simulink model "GenerateIPMSMCurrentProfile"  (R2026a)
settings: Solver=FixedStepAuto  StopTime=0.01  FixedStep=Ts
PreLoadFcn:
  | load('Model_Init.mat');
values from neighbouring files (symbols this model uses):
  BW = 750    [Model_Init.mat]
  idAxis = [-900 -882 -864 -846 -828 -810 -792 -774 -756 -738 -720 -702 ... (51 elements, 1x51)]    [Model_Init.mat]
  iqAxis = [0 17.3076923077 34.6153846154 51.9230769231 69.2307692308 86.5384615385 103.846153846 121.153846154 138.461538462 155.769230769 173.076923077 190.384615385 ... (53 elements, 1x53)]    [Model_Init.mat]
  Ki_d = 74.9060598039    [Model_Init.mat]
  Ki_q = 74.9060598039    [Model_Init.mat]
  lambdad = [-0.0631189178304 -0.0604505535566 -0.0577660230755 -0.0550656704567 -0.0523339959385 -0.0495630530333 -0.0467724011475 -0.043961149999 -0.041088360542 -0.0381850897745 -0.0352575152962 -0.0322924487897 ... (2703 elements, 51x53)]    [Model_Init.mat]
  lambdaq = [1.81058605777e-05 1.90263877371e-05 1.96027346878e-05 2.01239748193e-05 2.12091984783e-05 2.18705193678e-05 2.23125714149e-05 2.2585012385e-05 2.28163786723e-05 2.26620263018e-05 2.21885293033e-05 2.13315493573e-05 ... (2703 elements, 51x53)]    [Model_Init.mat]
  Ldd = [0.000148242459653 0.000148691520968 0.000149580086108 0.000150889642696 0.000152850483985 0.000154488744193 0.000155608417618 0.00015789001682 0.000160446117349 0.000161967923494 0.0001636844718 0.000166282231015 ... (2703 elements, 51x53)]    [Model_Init.mat]
  Lqq = [0.000400557309226 0.000405173323325 0.000409987177942 0.000414914340273 0.000419888602874 0.000424960583757 0.000430114747461 0.000435342158236 0.000440633705793 0.000446010815939 0.000451479502648 0.000457041392507 ... (2703 elements, 51x53)]    [Model_Init.mat]
  optimalTables =     [Model_Init.mat]
  PolePairs = 4    [Model_Init.mat]
  Ts = 1e-06    [Model_Init.mat]
  Tst = 0.0001    [Model_Init.mat]
undefined symbols (not defined in the file or in its folder): DiscIntNeverNeededParam
libraries: nesl_utility x13, fl_lib x7, ee_lib x5, eePwmGeneratorTwoLevel x1
settings Model: Creator=dakaihu  LastModifiedBy=dakaihu
settings SimscapeCC: SimscapeNominalValues="[{\"value\":\"1\",\"unit\":\"A\"},{\"value\":\"1\",\"unit\":\"bar\"},{\"value\":\"1\",\"unit\":\"cm^2\"},{\"value\":\"1\",\"unit\":\"cm^3/s\"},{\"value\":\"1\",\"unit\":\"kJ/kg\"},{\"value\":\"1\",\"unit\":\"kW\"},{\"value\":\"1\",\"unit\":\"l\"},{\"value\":\"1\",\"unit\":\"N\"},{\"value\":\"1\",\"unit\":\"N*m\"},{\"value\":\"1\",\"unit\":\"V\"}]"  SimscapeLogType=none  SimscapeLogDataHistory=5000.0

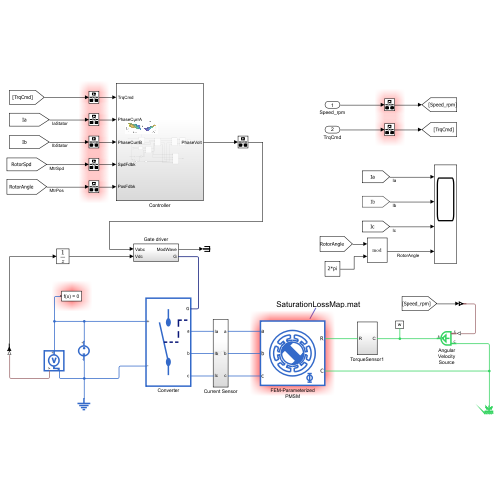
[thumbnail: Simulink's stored preview of the top-level diagram]
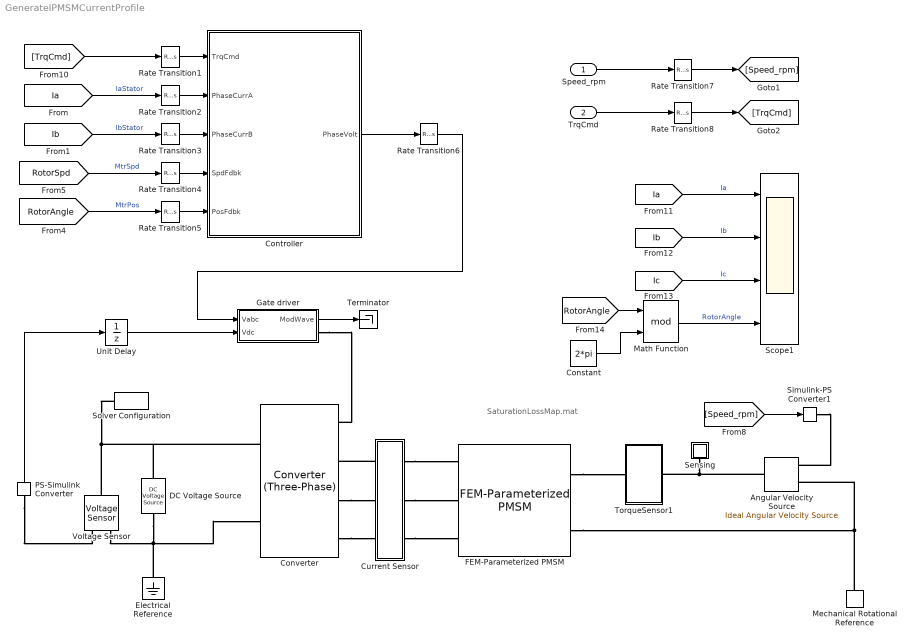
== system GenerateIPMSMCurrentProfile ==
  note: SaturationLossMap.mat
  Speed_rpm : Inport
  TrqCmd : Inport  Port=2
  Angular Velocity Source : fl_lib/Mechanical/Mechanical Sources/Ideal Angular Velocity Source
  Constant : Constant  Value=2*pi
  Controller : Subsystem
  Converter : ee_lib/Semiconductors & Converters/Converters/Converter (Three-Phase)  port_option=ee.enum.threePhasePort.expanded  fidelity_option=ee.enum.converters.fidelity.detailed  device_type=3  showThermalPort=false  K=0  Vth=0.5 V  Vgt=1 V  Vgt_off=-1 V  Ih=1 A  Vf=0.8 V  Ron=0.001 Ohm  Rds=0.001 Ohm  Goff=1e-5 1/Ohm  Eon_scalar=22.86e-3 J  Eoff_scalar=17.14e-3 J  Eoff_natural_commutation=10e-3 J  Voff=300 V  Iout_scalar=600 A  onCurrentMeasDelay=0 s  useCurrentFromPreviousCycle=false  useVoltageFromPreviousCycle=false  diode_param=2  diode_Vf=0.8 V  diode_Ron=0.001 Ohm  diode_Goff=1e-5 1/Ohm  diode_C=50 nF  diode_iRM=-235 A  diode_iF=300 A  diode_idot=-50 A/us  diode_trr_param=1  diode_trr_factor=3  diode_trr=15 us  diode_Qrr=1.5e+3 s*uA  diode_rec_loss_model=ee.enum.diode.reverseRecoveryModel.fixed  diode_ErecVal=0 J  diode_scaleWithIandV=false  diode_ErecMat=zeros(2, 3) J  diode_TjrecVec=[298.15, 398.15] K  diode_IfrecVec=[.1, 1, 10] A  diode_IrecVal=10 A  diode_VrecVal=10 V  diode_tFilter=1 / 1000 / 100 s  thermal_network_parameterization=ee.enum.thermalNetworkTopology.external  Rth=[.08, .5] K/W  Rth_Cauer=[.08, .1, .5] K/W  Rth_Foster=[.08, .14, .22, .16] K/W  thermal_mass_parameterization=ee.enum.thermalNetwork.timeconstant  thermal_mass=[.01, .5] J/K  thermal_mass_Cauer=[.01, .1, .5] J/K  thermal_mass_Foster=[.001, .005, .05, .5] J/K  thermal_time_constant=[.001, .2] s  thermal_time_constant_Cauer=[.001, .1, .2] s  thermal_time_constant_Foster=[7e-05, .0007, .01, .08] s  thermal_mass_initial_temperatures=[25, 25] degC  thermal_mass_initial_temperatures_Cauer=[25, 25, 25] degC  junction_thermal_mass=0.01 J/K  Tvec_initial_Foster=[25, 25, 25, 25] degC  snubber_type=0  Cs=1e-7 F  Rs=0.1 Ohm  Vce_loss=[0, 150, 300] V
  Current Sensor : Subsystem
  DC Voltage Source : ee_lib/Additional Components/SPICE Sources/DC Voltage Source  DC=720 V
  Electrical Reference : fl_lib/Electrical/Electrical Elements/Electrical Reference
  FEM-Parameterized PMSM : ee_lib/Electromechanical/Permanent Magnet/FEM-Parameterized PMSM  parameterization=1  winding_type=ee.enum.statorconnection.wye  iVec=[-2, 0, 2] A  xVec=[0, 20, 40, 60] deg  dfluxdiMatrix=0.0002 * ones(3, 4) Wb/A  dfluxdxMatrix=[0, -.16, .16, 0; 0, -.16, .16, 0; 0, -.16, .16, 0] Wb/rad  calculate_torque_matrix=1  TorqueMatrix=zeros(3, 3, 3, 4) N*m  idVec1=[-200, 0, 200] A  iqVec1=[-200, 0, 200] A  LdMatrix=0.0002 * ones(3, 3) H  LqMatrix=0.0002 * ones(3, 3) H  PmMatrix=0.1 * ones(3, 3) Wb  interp_method=simscape.enum.interpolation.linear  N=6  Rs=Rs Ohm  Ms=0.00002 H  L0=0.00016 H  loss_param=ee.enum.fem_motor.ironLossesExtended.empirical  losses_oc=[0, 0, 0] W  losses_sc=[0, 0, 0] W  f_losses=60 Hz  Isc_losses=95 A  Inertia=0 kg*m^2  lam=0 N*m/(rad/s)  i_d_specify=off  i_d_priority=None  i_d=0 A  i_d_nominal_specify=off  i_d_nominal_value=1  i_d_nominal_unit=A  i_q_specify=off  i_q_priority=None  i_q=0 A  i_q_nominal_specify=off  i_q_nominal_value=1  i_q_nominal_unit=A  torque_specify=off  torque_priority=None  torque=0 N*m  torque_nominal_specify=off  torque_nominal_value=1  torque_nominal_unit=N*m  angular_velocity_specify=on  angular_velocity_priority=Low  angular_velocity=1000 rpm  angular_velocity_nominal_specify=off  angular_velocity_nominal_value=1  angular_velocity_nominal_unit=rpm  angular_position_specify=off  angular_position_priority=High  angular_position=0 deg  angular_position_nominal_specify=off  angular_position_nominal_value=1  angular_position_nominal_unit=deg  alpha=3.93e-3 1/K  alpha_flux=-0.001 1/K  Tmeas=298.15 K  stator_thermal_mass=100 J/K  stator_initial_temperatures=[298.15, 298.15, 298.15] K  rotor_thermal_mass=200 J/K  rotor_initial_temperature=298.15 K  Rm_percent_rotor=90  Rd_percent_rotor=30  idVec=[-200, 0, 200] A  iqVec=[-200, 0, 200] A  dfluxAdiaMatrix3D=zeros(3, 3, 4) Wb/A  dfluxAdibMatrix3D=zeros(3, 3, 4) Wb/A  dfluxAdicMatrix3D=zeros(3, 3, 4) Wb/A  dfluxAdxMatrix3D=zeros(3, 3, 4) Wb/rad  TorqueMatrix3D=zeros(3, 3, 4) N*m  iaVec=[-200, 0, 200] A  ibVec=[-200, 0, 200] A  icVec=[-200, 0, 200] A  dfluxAdiaMatrix=zeros(3, 3, 3, 4) Wb/A  dfluxAdibMatrix=zeros(3, 3, 3, 4) Wb/A  dfluxAdicMatrix=zeros(3, 3, 3, 4) Wb/A  dfluxAdxMatrix=zeros(3, 3, 3, 4) Wb/rad  param_dq0=ee.enum.fem_motor.fluxTabulationOption.DQpolar  winding_type_dq0=1  expose_neutral_port=ee.enum.fem_motor.exposeNeutralPort.no  nPolePairs=PolePairs  parks_type=ee.enum.fem_motor.parksType.QleadsD_AphaseToQaxis  idVec2=idVec A  iqVec2=iqVec A  magVec2=MagVec A  betaVec2=gammaVec deg  xVec2=angleVec deg  fluxD_dq0=fluxD Wb  fluxQ_dq0=fluxQ Wb  fluxA_dq0=fluxAmat Wb  Torque_dq0=torque N*m  fluxD_IBX=Fd Wb  fluxQ_IBX=Fq Wb  fluxA_IBX=fluxAmat Wb  Torque_IBX=torqueMat N*m  rotorLossCoeff_k_h_DQ=zeros(3, 3) W/Hz  rotorLossCoeff_k_J_DQ=zeros(3, 3) W/Hz^2  rotorLossCoeff_k_ex_DQ=zeros(3, 3) W/Hz^1.50000  rotorLossCoeff_k_h_IB=zeros(3, 5) W/Hz  rotorLossCoeff_k_J_IB=zeros(3, 5) W/Hz^2  rotorLossCoeff_k_ex_IB=zeros(3, 5) W/Hz^1.50000  statorLossCoeff_k_h_DQ=zeros(3, 3) W/Hz  statorLossCoeff_k_J_DQ=zeros(3, 3) W/Hz^2  statorLossCoeff_k_ex_DQ=zeros(3, 3) W/Hz^1.50000  statorLossCoeff_k_h_IB=zeros(3, 5) W/Hz  statorLossCoeff_k_J_IB=zeros(3, 5) W/Hz^2  statorLossCoeff_k_ex_IB=zeros(3, 5) W/Hz^1.50000  wVec=[1000, 2000] rpm  rotorLossTable_DQ=zeros(3, 3, 2) W  statorLossTable_DQ=zeros(3, 3, 2) W  rotorLossTable_IB=zeros(3, 5, 2) W  statorLossTable_IB=zeros(3, 5, 2) W  electrical_torque_before_iron_losses_specify=off  electrical_torque_before_iron_losses_priority=None  electrical_torque_before_iron_losses=0 N*m  electrical_torque_before_iron_losses_nominal_specify=off  electrical_torque_before_iron_losses_nominal_value=1  electrical_torque_before_iron_losses_nominal_unit=N*m  Qrotor_specify=off  Qrotor_priority=None  Qrotor=0 J/s  Qrotor_nominal_specify=off  Qrotor_nominal_value=1  Qrotor_nominal_unit=J/s  Qstator_specify=off  Qstator_priority=None  Qstator=0 J/s  Qstator_nominal_specify=off  Qstator_nominal_value=1  Qstator_nominal_unit=J/s
  Gate driver : Subsystem
  Math Function : Math  Operator=mod
  Mechanical Rotational Reference : fl_lib/Mechanical/Rotational Elements/Mechanical Rotational Reference
  PS-Simulink Converter : nesl_utility/PS-Simulink Converter  PhysicalDomain=network_engine_domain  SubClassName=ps_output  LeftPortType=input  RightPortType=output  PseudoPeriodic=off  Frequencies=[]  VectorFormat=inherit  Unit=V  AffineConversion=off
  Rate Transition{1..5,7..8} (7 alike) : RateTransition  OutPortSampleTime=Tst
  Rate Transition6 : RateTransition
  Scope1 : Scope  NumInputPorts=4
      settings: ActiveDisplayYMinimum=-1.2392913585991725E-13  ActiveDisplayYMaximum=1.093469821040979E-12  DataLoggingVariableName=IPMSM_Currents  DataLoggingSaveFormat=Structure
  Sensing : Subsystem
      mask Display: disp('w');
  Simulink-PS Converter1 : nesl_utility/Simulink-PS Converter  PhysicalDomain=network_engine_domain  SubClassName=ps_input  LeftPortType=input  RightPortType=output  PseudoPeriodic=off  Frequencies=[]  NoiseDistribution=none  NoiseParameters=[]  Unit=rpm  AffineConversion=off  FilteringAndDerivatives=provide  SimscapeFilterOrder=1  InputFilterTimeConstant=0.001  UdotUserProvided=0
  Solver Configuration : nesl_utility/Solver Configuration  PhysicalDomain=network_engine_domain  SubClassName=solver  LeftPortType=input  RightPortType=generic  Tones=[]  Harmonics=[]  SimulateNoise=off  Profile=off  UseLocalSampling=off  EnableSwitchedLinearOptims=on  FrequencyDomain=off  UseCCode=off  RelTol=0.001  AbsTol=1e-06  MinStep=1e-09  ToWorkspace=off  RevertToSquareIcSolve=off  NumHomotopyIterations=100  PhasorMode=off  PhasorModeNumHarmonics=1  ConsistencySolver=NEWTON_FTOL  CanonicalOrdering=UNORDERED  OptimizeIntermediates=UNOPTIMIZED  IndexReductionMethod=DerivativeReplacement  DoDC=off  ResidualTolerance=1e-9  ConsistencyTolSource=GLOBAL  ConsistencyAbsTol=0.001  ConsistencyRelTol=0.001  ConsistencyTolFactor=0.001  UseLocalSolver=on  LocalSolverChoice=NE_BACKWARD_EULER_ADVANCER  ResolveIndetEquations=on  FunctionEvalNumThread=1  LocalSolverSampleTime=Ts  DoFixedCost=off  MaxNonlinIter=4  MaxModeIter=2  ComputeImpulses=off  ImpulseIterations=2  LinearAlgebra=auto  LinearAlgebraNumThread=0  EquationFormulation=NE_TIME_EF  DelaysMemoryBudget=1024  AutomaticFiltering=on  FilteringTimeConstant=0.001  PartitionStorageMethod=AS_NEEDED  PartitionMemoryBudget=1024  PartitionMethod=FAST  MultibodyUseLocalSolver=off  MultibodyLocalSolverChoice=ODE1  MultibodyLocalSolverSampleTime=0.001
  Terminator : Terminator
  TorqueSensor1 : Subsystem
  Unit Delay : UnitDelay  SampleTime=-1
  Voltage Sensor : fl_lib/Electrical/Electrical Sensors/Voltage Sensor
  wires:
  Controller/1(PhaseVolt) -> Rate Transition6/1
  [TrqCmd] -> Rate Transition1/1
  [Ia] -> Rate Transition2/1  "IaStator"
  [RotorSpd] -> Rate Transition4/1  "MtrSpd"
  [RotorAngle] -> Rate Transition5/1  "MtrPos"
  Rate Transition1/1 -> Controller/1(TrqCmd)
  Rate Transition2/1 -> Controller/2(PhaseCurrA)
  [Ib] -> Rate Transition3/1  "IbStator"
  Rate Transition3/1 -> Controller/3(PhaseCurrB)
  Rate Transition4/1 -> Controller/4(SpdFdbk)
  Rate Transition5/1 -> Controller/5(PosFdbk)
  Rate Transition6/1 -> Gate driver/1(Vabc)
  Unit Delay/1 -> Gate driver/2(Vdc)
  Gate driver/1(ModWave) -> Terminator/1
  [Speed_rpm] -> Simulink-PS Converter1/1
  PS-Simulink Converter/1 -> Unit Delay/1
  Rate Transition7/1 -> [Speed_rpm]
  Rate Transition8/1 -> [TrqCmd]
  [RotorAngle] -> Math Function/1
  Constant/1 -> Math Function/2
  [Ia] -> Scope1/1  "Ia"
  [Ib] -> Scope1/2  "Ib"
  [Ic] -> Scope1/3  "Ic"
  Math Function/1 -> Scope1/4  "RotorAngle"
  Speed_rpm/1 -> Rate Transition7/1
  TrqCmd/1 -> Rate Transition8/1
  connections:
  Sensing/LConn1 -- Angular Velocity Source/LConn1 -- TorqueSensor1/RConn1
  Mechanical Rotational Reference/LConn1 -- Angular Velocity Source/RConn2 -- FEM-Parameterized PMSM/RConn2
  Solver Configuration/RConn1 -- Converter/RConn1 -- DC Voltage Source/LConn1 -- Voltage Sensor/LConn1
  Electrical Reference/LConn1 -- Converter/RConn2 -- DC Voltage Source/RConn1 -- Voltage Sensor/RConn2
  Gate driver/RConn1 -- Converter/LConn1
  Current Sensor/LConn1 -- Converter/LConn2
  Current Sensor/RConn1 -- FEM-Parameterized PMSM/LConn1
  Converter/LConn3 -- Current Sensor/LConn2
  Current Sensor/RConn2 -- FEM-Parameterized PMSM/LConn2
  Converter/LConn4 -- Current Sensor/LConn3
  Current Sensor/RConn3 -- FEM-Parameterized PMSM/LConn3
  Simulink-PS Converter1/RConn1 -- Angular Velocity Source/RConn1
  PS-Simulink Converter/LConn1 -- Voltage Sensor/RConn1
  FEM-Parameterized PMSM/RConn1 -- TorqueSensor1/LConn1

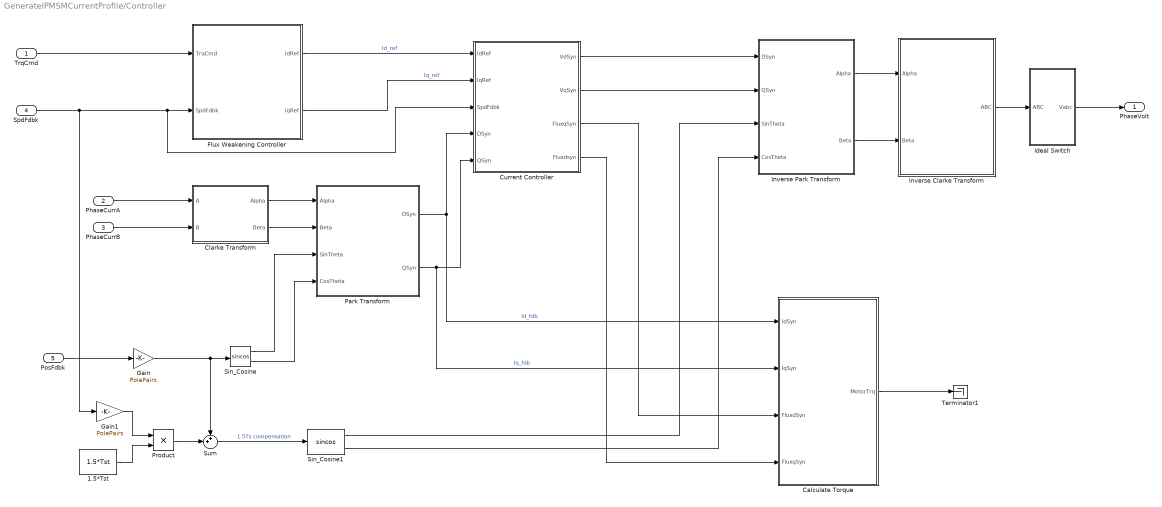
== system GenerateIPMSMCurrentProfile/Controller ==
  TrqCmd : Inport  OutDataTypeStr=double  PortDimensions=1  SampleTime=Tst
  PhaseCurrA : Inport  Port=2  OutDataTypeStr=double  PortDimensions=1  SampleTime=Tst
  PhaseCurrB : Inport  Port=3  OutDataTypeStr=double  PortDimensions=1  SampleTime=Tst
  SpdFdbk : Inport  Port=4  OutDataTypeStr=double  PortDimensions=1  SampleTime=Tst
  PosFdbk : Inport  Port=5  OutDataTypeStr=double  PortDimensions=1  SampleTime=Tst
  1.5*Tst : Constant  Value=1.5*Tst  SampleTime=-1
  Calculate Torque : Subsystem
  Clarke Transform : Subsystem
  Current Controller : Subsystem
  Flux Weakening Controller : Subsystem
  Gain : Gain  Gain=PolePairs
  Gain1 : Gain  Gain=PolePairs
  Ideal Switch : Subsystem  VariantControl=SpaceVectorModulation_JB
  Inverse Clarke Transform : Subsystem
  Inverse Park Transform : Subsystem
  Park Transform : Subsystem
  Product : Product
  Sin_Cosine : Trigonometry  Operator=sincos
  Sin_Cosine1 : Trigonometry  Operator=sincos
  Sum : Sum  Inputs=++|
  Terminator1 : Terminator
  PhaseVolt : Outport  OutDataTypeStr=double  Unit=V  PortDimensions=3  SampleTime=Tst  VectorParamsAs1DForOutWhenUnconnected=off
  wires:
  Flux Weakening Controller/1(IdRef) -> Current Controller/1(IdRef)  "Id_ref"
  SpdFdbk/1 -> Gain1/1, Current Controller/3(SpdFdbk), Flux Weakening Controller/2(SpdFdbk)
  Gain1/1 -> Product/1
  Sum/1 -> Sin_Cosine1/1  "1.5Ts compensation"
  Clarke Transform/1(Alpha) -> Park Transform/1(Alpha)
  Clarke Transform/2(Beta) -> Park Transform/2(Beta)
  Current Controller/1(VdSyn) -> Inverse Park Transform/1(DSyn)
  Inverse Park Transform/1(Alpha) -> Inverse Clarke Transform/1(Alpha)
  Sin_Cosine/1 -> Park Transform/3(SinTheta)
  Park Transform/2(QSyn) -> Current Controller/5(QSyn), Calculate Torque/2(IqSyn)  "Iq_fdb"
  Product/1 -> Sum/2
  Sin_Cosine/2 -> Park Transform/4(CosTheta)
  1.5*Tst/1 -> Product/2
  Calculate Torque/1(MotorTrq) -> Terminator1/1
  Current Controller/2(VqSyn) -> Inverse Park Transform/2(QSyn)
  Current Controller/3(FluxqSyn) -> Calculate Torque/3(FluxdSyn)
  Inverse Clarke Transform/1(ABC) -> Ideal Switch/1(ABC)
  PosFdbk/1 -> Gain/1
  Inverse Park Transform/2(Beta) -> Inverse Clarke Transform/2(Beta)
  Gain/1 -> Sum/1, Sin_Cosine/1
  PhaseCurrB/1 -> Clarke Transform/2(B)
  Park Transform/1(DSyn) -> Current Controller/4(DSyn), Calculate Torque/1(IdSyn)  "Id_fdb"
  TrqCmd/1 -> Flux Weakening Controller/1(TrqCmd)
  Current Controller/4(Fluxdsyn) -> Calculate Torque/4(FluxqSyn)
  Flux Weakening Controller/2(IqRef) -> Current Controller/2(IqRef)  "Iq_ref"
  Sin_Cosine1/2 -> Inverse Park Transform/4(CosTheta)
  Sin_Cosine1/1 -> Inverse Park Transform/3(SinTheta)
  PhaseCurrA/1 -> Clarke Transform/1(A)
  Ideal Switch/1(Vabc) -> PhaseVolt/1

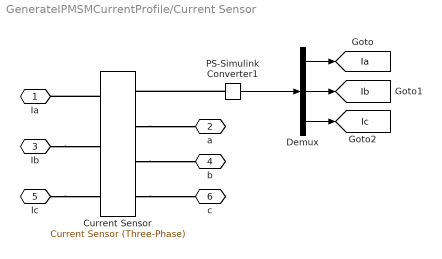
== system GenerateIPMSMCurrentProfile/Current Sensor ==
  Current Sensor : ee_lib/Sensors & Transducers/Current Sensor (Three-Phase)  port_option=ee.enum.threePhasePort.expanded
  Demux : Demux  Outputs=3
  PS-Simulink Converter1 : nesl_utility/PS-Simulink Converter  PhysicalDomain=network_engine_domain  SubClassName=ps_output  LeftPortType=input  RightPortType=output  PseudoPeriodic=off  Frequencies=[]  VectorFormat=inherit  Unit=A  AffineConversion=off
  Ia : PMIOPort  Side=Left
  a : PMIOPort  Port=2  Side=Right
  Ib : PMIOPort  Port=3  Side=Left
  b : PMIOPort  Port=4  Side=Right
  Ic : PMIOPort  Port=5  Side=Left
  c : PMIOPort  Port=6  Side=Right
  tag scope: Ia=global, Ib=global, Ic=global
  wires:
  Demux/1 -> [Ia]
  Demux/2 -> [Ib]
  Demux/3 -> [Ic]
  PS-Simulink Converter1/1 -> Demux/1
  connections:
  Current Sensor/RConn3 -- b/RConn1
  Ib/RConn1 -- Current Sensor/LConn2
  Current Sensor/RConn2 -- a/RConn1
  Current Sensor/LConn1 -- Ia/RConn1
  Current Sensor/RConn4 -- c/RConn1
  Ic/RConn1 -- Current Sensor/LConn3
  PS-Simulink Converter1/LConn1 -- Current Sensor/RConn1

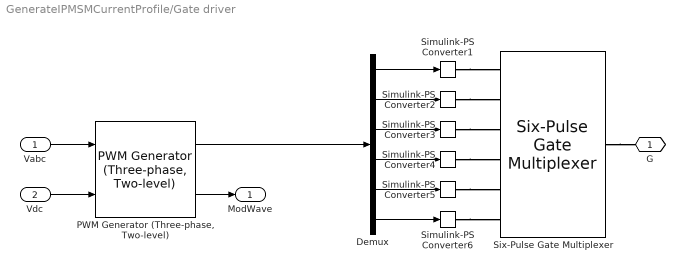
== system GenerateIPMSMCurrentProfile/Gate driver ==
  Vabc : Inport
  Vdc : Inport  Port=2
  Demux : Demux  Outputs=6
  "PWM Generator (Three-phase, Two-level)" : eePwmGeneratorTwoLevel/PWM Generator (Three-phase, Two-level)  PWMMode=Continuous PWM (CPWM)  CPWMMode=SVM: space vector modulation  DPWMMode=60 DPWM: 60 degree discontinuous PWM  fsw=1e4  Ts=Ts
  Simulink-PS Converter{1..6} (6 alike) : nesl_utility/Simulink-PS Converter  PhysicalDomain=network_engine_domain  SubClassName=ps_input  LeftPortType=input  RightPortType=output  PseudoPeriodic=off  Frequencies=[]  NoiseDistribution=none  NoiseParameters=[]  Unit=1  AffineConversion=off  FilteringAndDerivatives=zero  SimscapeFilterOrder=1  InputFilterTimeConstant=0.001  UdotUserProvided=1
  Six-Pulse Gate Multiplexer : ee_lib/Semiconductors & Converters/Converters/Six-Pulse Gate Multiplexer  port_option=ee.enum.controlport.ps
  G : PMIOPort  Side=Right
  ModWave : Outport
  wires:
  Demux/2 -> Simulink-PS Converter2/1
  Demux/3 -> Simulink-PS Converter3/1
  Demux/4 -> Simulink-PS Converter4/1
  Demux/6 -> Simulink-PS Converter6/1
  Demux/5 -> Simulink-PS Converter5/1
  "PWM Generator (Three-phase, Two-level)"/1 -> Demux/1
  Demux/1 -> Simulink-PS Converter1/1
  "PWM Generator (Three-phase, Two-level)"/2 -> ModWave/1
  Vdc/1 -> "PWM Generator (Three-phase, Two-level)"/2
  Vabc/1 -> "PWM Generator (Three-phase, Two-level)"/1
  connections:
  Simulink-PS Converter4/RConn1 -- Six-Pulse Gate Multiplexer/LConn4
  Simulink-PS Converter3/RConn1 -- Six-Pulse Gate Multiplexer/LConn3
  Simulink-PS Converter2/RConn1 -- Six-Pulse Gate Multiplexer/LConn2
  Simulink-PS Converter6/RConn1 -- Six-Pulse Gate Multiplexer/LConn6
  Simulink-PS Converter5/RConn1 -- Six-Pulse Gate Multiplexer/LConn5
  Simulink-PS Converter1/RConn1 -- Six-Pulse Gate Multiplexer/LConn1
  Six-Pulse Gate Multiplexer/RConn1 -- G/RConn1

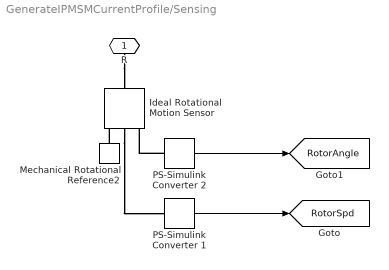
== system GenerateIPMSMCurrentProfile/Sensing ==
  Ideal Rotational Motion Sensor : fl_lib/Mechanical/Mechanical Sensors/Ideal Rotational Motion Sensor  reference=foundation.enum.MeasurementReference.difference  acceleration_port=false  velocity_port=true  position_port=true  wrap_angle=simscape.enum.onoff.off  offset=0 rad
  Mechanical Rotational Reference2 : fl_lib/Mechanical/Rotational Elements/Mechanical Rotational Reference
  PS-Simulink Converter 1 : nesl_utility/PS-Simulink Converter  PhysicalDomain=network_engine_domain  SubClassName=ps_output  LeftPortType=input  RightPortType=output  PseudoPeriodic=off  Frequencies=[]  VectorFormat=1-D array  Unit=rad/s  AffineConversion=off
  PS-Simulink Converter 2 : nesl_utility/PS-Simulink Converter  PhysicalDomain=network_engine_domain  SubClassName=ps_output  LeftPortType=input  RightPortType=output  PseudoPeriodic=off  Frequencies=[]  VectorFormat=1-D array  Unit=rad  AffineConversion=off
  R : PMIOPort  Side=Left
  tag scope: RotorAngle=global, RotorSpd=global
  wires:
  PS-Simulink Converter 1/1 -> [RotorSpd]
  PS-Simulink Converter 2/1 -> [RotorAngle]
  connections:
  Ideal Rotational Motion Sensor/RConn2 -- PS-Simulink Converter 1/LConn1
  Mechanical Rotational Reference2/LConn1 -- Ideal Rotational Motion Sensor/RConn1
  R/RConn1 -- Ideal Rotational Motion Sensor/LConn1
  PS-Simulink Converter 2/LConn1 -- Ideal Rotational Motion Sensor/RConn3

== system GenerateIPMSMCurrentProfile/TorqueSensor1 ==
  Goto11 : Goto  Commented=on  GotoTag=MotorTrq  TagVisibility=global
  Ideal Torque Sensor1 : fl_lib/Mechanical/Mechanical Sensors/Ideal Torque Sensor
  PS-Simulink Converter1 : nesl_utility/PS-Simulink Converter  PhysicalDomain=network_engine_domain  SubClassName=ps_output  LeftPortType=input  RightPortType=output  PseudoPeriodic=off  Frequencies=[]  VectorFormat=inherit  Unit=N*m  AffineConversion=off
  R : PMIOPort  Side=Left
  C : PMIOPort  Port=2  Side=Right
  wires:
  PS-Simulink Converter1/1 -> Goto11/1
  connections:
  Ideal Torque Sensor1/RConn2 -- PS-Simulink Converter1/LConn1
  R/RConn1 -- Ideal Torque Sensor1/LConn1
  C/RConn1 -- Ideal Torque Sensor1/RConn1

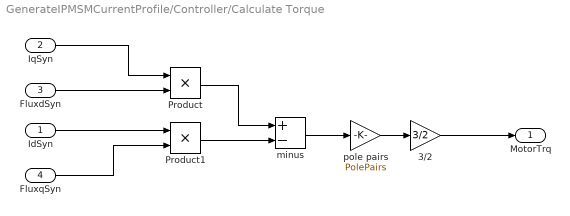
== system GenerateIPMSMCurrentProfile/Controller/Calculate Torque ==
  IdSyn : Inport
  IqSyn : Inport  Port=2
  FluxdSyn : Inport  Port=3
  FluxqSyn : Inport  Port=4
  3/2 : Gain  Gain=3/2
  Product : Product
  Product1 : Product
  minus : Sum  Inputs=+-
  pole pairs : Gain  Gain=PolePairs
  MotorTrq : Outport  VectorParamsAs1DForOutWhenUnconnected=off
  wires:
  FluxqSyn/1 -> Product1/2
  FluxdSyn/1 -> Product/2
  pole pairs/1 -> 3/2/1
  IdSyn/1 -> Product1/1
  IqSyn/1 -> Product/1
  Product/1 -> minus/1
  minus/1 -> pole pairs/1
  Product1/1 -> minus/2
  3/2/1 -> MotorTrq/1

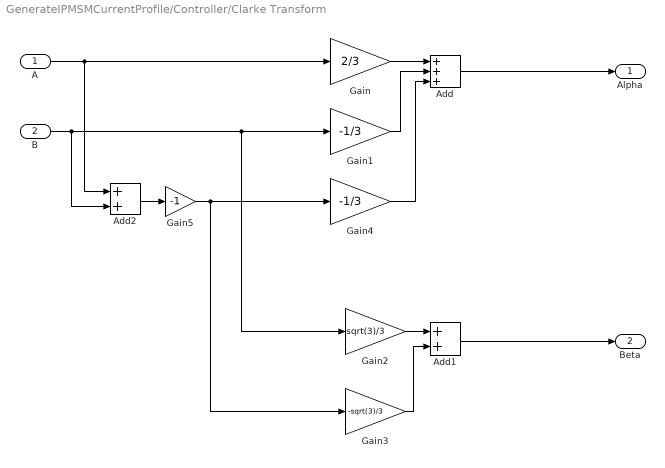
== system GenerateIPMSMCurrentProfile/Controller/Clarke Transform ==
  A : Inport
  B : Inport  Port=2
  Add : Sum  Inputs=+++
  Add1 : Sum
  Add2 : Sum
  Gain : Gain  Gain=2/3
  Gain1 : Gain  Gain=-1/3
  Gain2 : Gain  Gain=sqrt(3)/3
  Gain3 : Gain  Gain=-sqrt(3)/3
  Gain4 : Gain  Gain=-1/3
  Gain5 : Gain  Gain=-1
  Alpha : Outport  VectorParamsAs1DForOutWhenUnconnected=off
  Beta : Outport  Port=2  VectorParamsAs1DForOutWhenUnconnected=off
  wires:
  Gain5/1 -> Gain3/1, Gain4/1
  A/1 -> Gain/1, Add2/1
  Gain/1 -> Add/1
  B/1 -> Gain2/1, Gain1/1, Add2/2
  Gain1/1 -> Add/2
  Add/1 -> Alpha/1
  Add1/1 -> Beta/1
  Gain2/1 -> Add1/1
  Add2/1 -> Gain5/1
  Gain3/1 -> Add1/2
  Gain4/1 -> Add/3

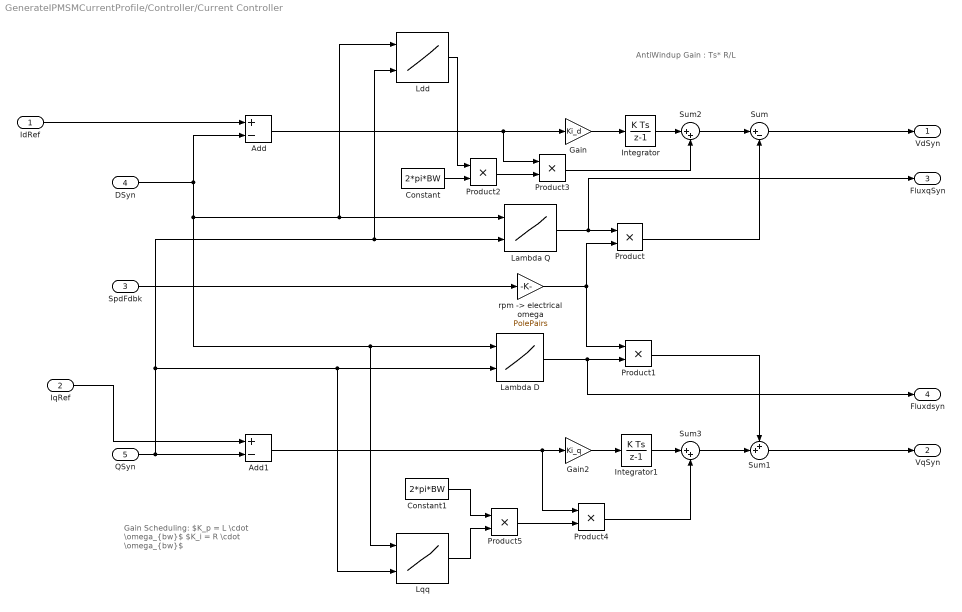
== system GenerateIPMSMCurrentProfile/Controller/Current Controller ==
  note: AntiWindup Gain : Ts* R/L
  note: Gain Scheduling:
      | $K_p = L \cdot \omega_{bw}$
      | $K_i = R \cdot \omega_{bw}$
  IdRef : Inport
  IqRef : Inport  Port=2
  SpdFdbk : Inport  Port=3
  DSyn : Inport  Port=4
  QSyn : Inport  Port=5
  Add : Sum  Inputs=+-
  Add1 : Sum  Inputs=+-
  Constant : Constant  Value=2*pi*BW  SampleTime=-1
  Constant1 : Constant  Value=2*pi*BW  SampleTime=-1
  Gain : Gain  Gain=Ki_d
  Gain2 : Gain  Gain=Ki_q
  Integrator : DiscreteIntegrator  SampleTime=-1  ICPrevOutput=DiscIntNeverNeededParam  ICPrevScaledInput=DiscIntNeverNeededParam
  Integrator1 : DiscreteIntegrator  SampleTime=-1  ICPrevOutput=DiscIntNeverNeededParam  ICPrevScaledInput=DiscIntNeverNeededParam
  Lambda D : Lookup_n-D  BreakpointsForDimension1=idAxis  BreakpointsForDimension2=iqAxis  BreakpointsForDimension3=[5, 7]  Table=lambdad  InternalRulePriority=Speed  RndMeth=Simplest
      settings: InputPortMap=u0,u1
  Lambda Q : Lookup_n-D  BreakpointsForDimension1=idAxis  BreakpointsForDimension2=iqAxis  BreakpointsForDimension3=[5, 7]  Table=lambdaq  InternalRulePriority=Speed  RndMeth=Simplest
      settings: InputPortMap=u0,u1
  Ldd : Lookup_n-D  BreakpointsForDimension1=idAxis  BreakpointsForDimension2=iqAxis  BreakpointsForDimension3=[5, 7]  Table=Ldd  InternalRulePriority=Speed  RndMeth=Simplest
      settings: InputPortMap=u0,u1
  Lqq : Lookup_n-D  BreakpointsForDimension1=idAxis  BreakpointsForDimension2=iqAxis  BreakpointsForDimension3=[5, 7]  Table=Lqq  InternalRulePriority=Speed  RndMeth=Simplest
      settings: InputPortMap=u0,u1
  Product{,1..5} (6 alike) : Product
  Sum : Sum  Inputs=|+-
  Sum1 : Sum  Inputs=++|
  Sum2 : Sum  Inputs=|++
  Sum3 : Sum  Inputs=|++
  "rpm -> electrical omega" : Gain  Gain=PolePairs
  VdSyn : Outport  VectorParamsAs1DForOutWhenUnconnected=off
  VqSyn : Outport  Port=2  VectorParamsAs1DForOutWhenUnconnected=off
  FluxqSyn : Outport  Port=3  VectorParamsAs1DForOutWhenUnconnected=off
  Fluxdsyn : Outport  Port=4  VectorParamsAs1DForOutWhenUnconnected=off
  wires:
  Add1/1 -> Product4/1, Gain2/1
  Sum3/1 -> Sum1/2
  Product4/1 -> Sum3/2
  Gain2/1 -> Integrator1/1
  Integrator1/1 -> Sum3/1
  Sum2/1 -> Sum/1
  Add/1 -> Product3/1, Gain/1
  Product3/1 -> Sum2/2
  Integrator/1 -> Sum2/1
  Gain/1 -> Integrator/1
  Sum1/1 -> VqSyn/1
  Sum/1 -> VdSyn/1
  Product1/1 -> Sum1/1
  Lambda D/1 -> Product1/2, Fluxdsyn/1
  DSyn/1 -> Add/2, Ldd/1, Lambda Q/1, Lambda D/1, Lqq/1
  QSyn/1 -> Add1/2, Lqq/2, Lambda D/2, Ldd/2, Lambda Q/2
  "rpm -> electrical omega"/1 -> Product/2, Product1/1
  Lambda Q/1 -> Product/1, FluxqSyn/1
  IqRef/1 -> Add1/1
  SpdFdbk/1 -> "rpm -> electrical omega"/1
  IdRef/1 -> Add/1
  Ldd/1 -> Product2/1
  Constant/1 -> Product2/2
  Product2/1 -> Product3/2
  Product5/1 -> Product4/2
  Constant1/1 -> Product5/1
  Lqq/1 -> Product5/2
  Product/1 -> Sum/2

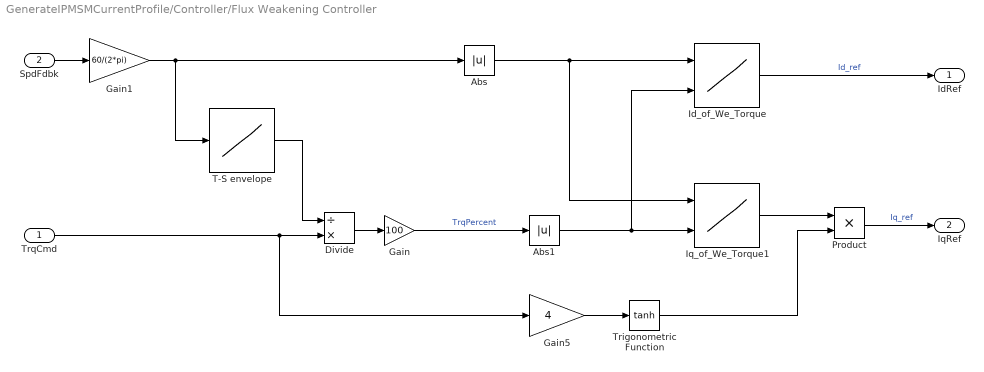
== system GenerateIPMSMCurrentProfile/Controller/Flux Weakening Controller ==
  TrqCmd : Inport
  SpdFdbk : Inport  Port=2
  Abs : Abs  SaturateOnIntegerOverflow=off
  Abs1 : Abs  SaturateOnIntegerOverflow=off
  Divide : Product  Inputs=/*
  Gain : Gain  Gain=100
  Gain1 : Gain  Gain=60/(2*pi)
  Gain5 : Gain  Gain=4  SaturateOnIntegerOverflow=on  OutDataTypeStr=Inherit: Same as input  ParamDataTypeStr=Inherit: Same as input
  Id_of_We_Torque : Lookup_n-D  BreakpointsForDimension1=optimalTables.n_norm  BreakpointsForDimension2=optimalTables.TrqPercent_norm  Table=optimalTables.Id_Table  ExtrapMethod=Clip  UseLastTableValue=on  InternalRulePriority=Speed  RndMeth=Simplest
      settings: InputPortMap=u0,u1
  Iq_of_We_Torque1 : Lookup_n-D  BreakpointsForDimension1=optimalTables.n_norm  BreakpointsForDimension2=optimalTables.TrqPercent_norm  Table=optimalTables.Iq_Table  ExtrapMethod=Clip  UseLastTableValue=on  InternalRulePriority=Speed  RndMeth=Simplest
      settings: InputPortMap=u0,u1
  Product : Product
  T-S envelope : Lookup_n-D  NumberOfTableDimensions=1  BreakpointsForDimension1=optimalTables.n_norm  Table=optimalTables.TrqEnvelope  InternalRulePriority=Speed  RndMeth=Simplest
  Trigonometric Function : Trigonometry  Operator=tanh
  IdRef : Outport  VectorParamsAs1DForOutWhenUnconnected=off
  IqRef : Outport  Port=2  VectorParamsAs1DForOutWhenUnconnected=off
  wires:
  Gain5/1 -> Trigonometric Function/1
  Abs1/1 -> Id_of_We_Torque/2, Iq_of_We_Torque1/2
  Product/1 -> IqRef/1  "Iq_ref"
  Trigonometric Function/1 -> Product/2
  Iq_of_We_Torque1/1 -> Product/1
  Abs/1 -> Id_of_We_Torque/1, Iq_of_We_Torque1/1
  Id_of_We_Torque/1 -> IdRef/1  "Id_ref"
  TrqCmd/1 -> Gain5/1, Divide/2
  SpdFdbk/1 -> Gain1/1
  T-S envelope/1 -> Divide/1
  Divide/1 -> Gain/1
  Gain/1 -> Abs1/1  "TrqPercent"
  Gain1/1 -> T-S envelope/1, Abs/1

== system GenerateIPMSMCurrentProfile/Controller/Ideal Switch ==
  ABC : Inport
  Vabc : Outport  VectorParamsAs1DForOutWhenUnconnected=off
  wires:
  ABC/1 -> Vabc/1

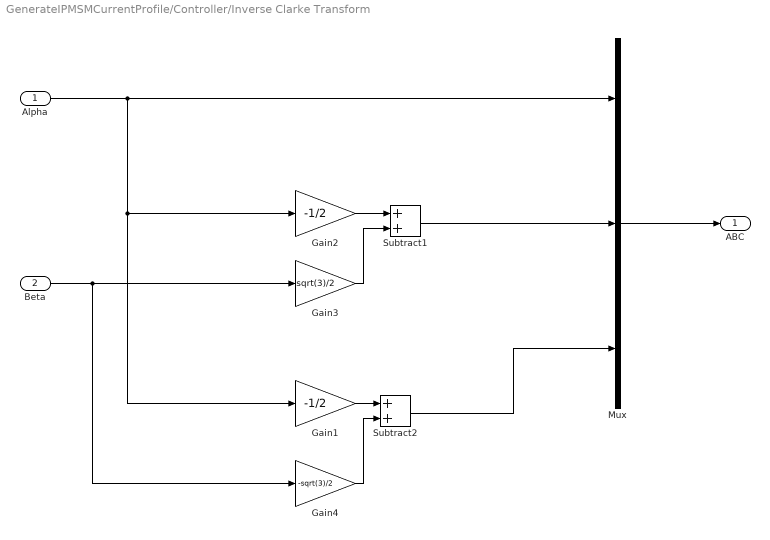
== system GenerateIPMSMCurrentProfile/Controller/Inverse Clarke Transform ==
  Alpha : Inport
  Beta : Inport  Port=2
  Gain1 : Gain  Gain=-1/2
  Gain2 : Gain  Gain=-1/2
  Gain3 : Gain  Gain=sqrt(3)/2
  Gain4 : Gain  Gain=-sqrt(3)/2
  Mux : Mux  Inputs=3
  Subtract1 : Sum
  Subtract2 : Sum
  ABC : Outport  VectorParamsAs1DForOutWhenUnconnected=off
  wires:
  Mux/1 -> ABC/1
  Gain3/1 -> Subtract1/2
  Gain2/1 -> Subtract1/1
  Subtract1/1 -> Mux/2
  Alpha/1 -> Gain2/1, Gain1/1, Mux/1
  Beta/1 -> Gain4/1, Gain3/1
  Subtract2/1 -> Mux/3
  Gain4/1 -> Subtract2/2
  Gain1/1 -> Subtract2/1

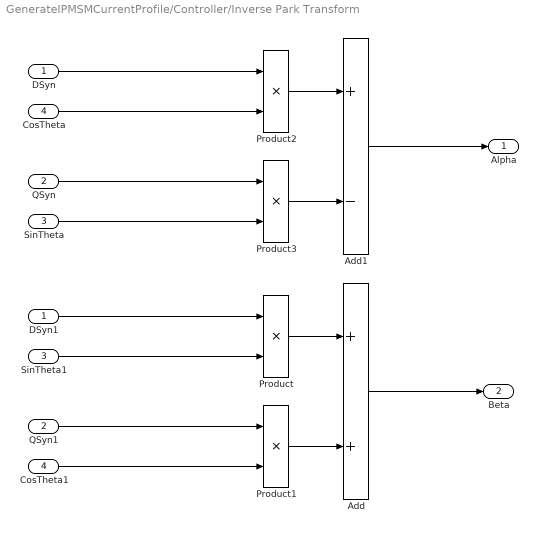
== system GenerateIPMSMCurrentProfile/Controller/Inverse Park Transform ==
  DSyn : Inport
  QSyn : Inport  Port=2
  SinTheta : Inport  Port=3
  CosTheta : Inport  Port=4
  Add : Sum
  Add1 : Sum  Inputs=+-
  CosTheta1 : InportShadow  Port=4
  DSyn1 : InportShadow
  Product{,1..3} (4 alike) : Product  RndMeth=Zero
  QSyn1 : InportShadow  Port=2
  SinTheta1 : InportShadow  Port=3
  Alpha : Outport  VectorParamsAs1DForOutWhenUnconnected=off
  Beta : Outport  Port=2  VectorParamsAs1DForOutWhenUnconnected=off
  wires:
  Product/1 -> Add/1
  Product1/1 -> Add/2
  Add/1 -> Beta/1
  Product2/1 -> Add1/1
  Product3/1 -> Add1/2
  Add1/1 -> Alpha/1
  DSyn1/1 -> Product/1
  SinTheta1/1 -> Product/2
  CosTheta1/1 -> Product1/2
  QSyn1/1 -> Product1/1
  CosTheta/1 -> Product2/2
  QSyn/1 -> Product3/1
  SinTheta/1 -> Product3/2
  DSyn/1 -> Product2/1

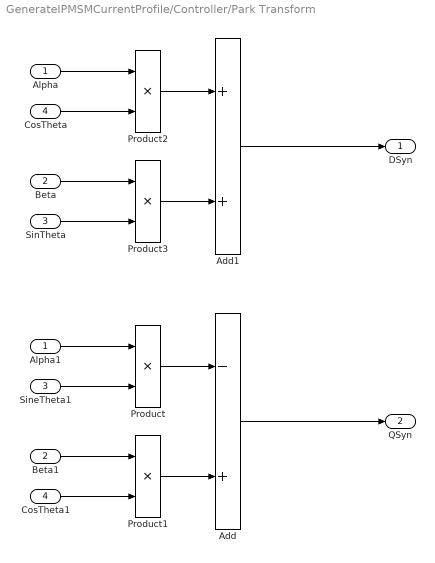
== system GenerateIPMSMCurrentProfile/Controller/Park Transform ==
  Alpha : Inport
  Beta : Inport  Port=2
  SinTheta : Inport  Port=3
  CosTheta : Inport  Port=4
  Add : Sum  Inputs=-+
  Add1 : Sum
  Alpha1 : InportShadow
  Beta1 : InportShadow  Port=2
  CosTheta1 : InportShadow  Port=4
  Product{,1..3} (4 alike) : Product  RndMeth=Zero
  SineTheta1 : InportShadow  Port=3
  DSyn : Outport  VectorParamsAs1DForOutWhenUnconnected=off
  QSyn : Outport  Port=2  VectorParamsAs1DForOutWhenUnconnected=off
  wires:
  CosTheta1/1 -> Product1/2
  SineTheta1/1 -> Product/2
  SinTheta/1 -> Product3/2
  CosTheta/1 -> Product2/2
  Beta/1 -> Product3/1
  Alpha/1 -> Product2/1
  Beta1/1 -> Product1/1
  Alpha1/1 -> Product/1
  Add1/1 -> DSyn/1
  Product3/1 -> Add1/2
  Product2/1 -> Add1/1
  Add/1 -> QSyn/1
  Product1/1 -> Add/2
  Product/1 -> Add/1
